simulink model "SIXDOF28"  (R2025b)
settings: Solver=VariableStepAuto  StartTime=0.0  StopTime=sortieStopTime_s  MaxStep=2.0  RelTol=1e-3
undefined symbols (not defined in the file): aircraft_mass, alpha0, alpha_bp, b, CL_table, ClCsurfaces, Cldampingrates, Cldeltae, CmCsurfaces, Cmdampingrates, CnCsurfaces, Cndampingrates, COP, CruiseSpeed, deg, density, DiscIntNeverNeededParam, dwGrad, ElTrim, g, h0, InitialHeadingRadBySortie, InitialPosBySortie, InitPitch, InitUb, Initwb, l, lt, maxPropRad, payloadvolume, PitchTrim, rad, rho, s, S, selectedSortie, St, ThrottleTrim
libraries: slpidlib x12, aerolibasang x3, aerolibconvert2 x2, aerolibadyn x1
(part 3 of 3)

== matlab function SIXDOF28/Subsystem2/Spraying/MATLAB Function2 ==
  settings: updateMethod=DISCRETE
  data: currentPosNED input; sprayActive output; sprayWaypointsNED input; activeSprayLaneIdx output; startGateHit output; endGateHit output; crossTrackToLane_m output; alongTrack_m output; heightError_m output; gateState output; inStartGate output; inEndGate output
function [sprayActive, activeSprayLaneIdx, startGateHit, endGateHit, ...
    crossTrackToLane_m, alongTrack_m, heightError_m, gateState, ...
    inStartGate, inEndGate] = sprayGateLogicNED(currentPosNED, sprayWaypointsNED)
%#codegen
% sprayGateLogicNED
% Simulink-friendly spray on/off logic using rectangular start/end gates
% built from spray-lane start/end waypoint pairs in NED coordinates.
%
% Inputs:
%   currentPosNED      [1x3] or [3x1] vehicle position [North East Down] [m]
%   sprayWaypointsNED  [2*N x 3] spray-lane waypoint pairs:
%                      [start1; end1; start2; end2; ...]
%
% Outputs:
%   sprayActive          1 while spraying on the active lane, else 0
%   activeSprayLaneIdx   current spray lane index being armed or sprayed
%   startGateHit         1 on the sample when the start gate is crossed
%   endGateHit           1 on the sample when the end gate is crossed
%   crossTrackToLane_m   signed horizontal cross-track error to active lane [m]
%   alongTrack_m         along-track position on active lane from lane start [m]
%   heightError_m        vertical error to closest point on active lane [m]
%   gateState            0 waiting for start gate, 1 spraying, 2 complete
%   inStartGate          1 when current position is inside the start gate box
%   inEndGate            1 when current position is inside the end gate box
%
% Gate geometry assumptions:
% - Start and end gates are rectangles perpendicular to the lane direction.
% - Gate width is 10 m total (5 m either side of the lane centreline).
% - Gate thickness is 2 m along the lane direction.
% - Gate height is 2 m total around the planned waypoint altitude.
% - Spray turns on when the aircraft crosses the start gate in the correct
%   direction and within the gate bounds.
% - Spray turns off when the aircraft crosses the end gate in the correct
%   direction and within the gate bounds.

    persistent laneIdxPersistent sprayOnPersistent ...
        previousPosPersistent hasPreviousPosPersistent ...
        previousWaypointCount previousFirstNorth previousFirstEast previousFirstDown ...
        previousLastNorth previousLastEast previousLastDown

    pos = zeros(1,3);
    pos(1) = currentPosNED(1);
    pos(2) = currentPosNED(2);
    pos(3) = currentPosNED(3);

    sprayActive = 0.0;
    activeSprayLaneIdx = 1.0;
    startGateHit = 0.0;
    endGateHit = 0.0;
    crossTrackToLane_m = 0.0;
    alongTrack_m = 0.0;
    heightError_m = 0.0;
    gateState = 0.0;
    inStartGate = 0.0;
    inEndGate = 0.0;

    waypointCount = size(sprayWaypointsNED, 1);
    if waypointCount < 2 || size(sprayWaypointsNED, 2) < 3
        return
    end

    laneCount = floor(waypointCount / 2);
    if laneCount < 1
        return
    end

    if isempty(laneIdxPersistent)
        laneIdxPersistent = 1;
        sprayOnPersistent = false;
        previousPosPersistent = pos;
        hasPreviousPosPersistent = false;
        previousWaypointCount = waypointCount;
        previousFirstNorth = sprayWaypointsNED(1,1);
        previousFirstEast = sprayWaypointsNED(1,2);
        previousFirstDown = sprayWaypointsNED(1,3);
        previousLastNorth = sprayWaypointsNED(waypointCount,1);
        previousLastEast = sprayWaypointsNED(waypointCount,2);
        previousLastDown = sprayWaypointsNED(waypointCount,3);
    end

    if previousWaypointCount ~= waypointCount || ...
            previousFirstNorth ~= sprayWaypointsNED(1,1) || ...
            previousFirstEast ~= sprayWaypointsNED(1,2) || ...
            previousFirstDown ~= sprayWaypointsNED(1,3) || ...
            previousLastNorth ~= sprayWaypointsNED(waypointCount,1) || ...
            previousLastEast ~= sprayWaypointsNED(waypointCount,2) || ...
            previousLastDown ~= sprayWaypointsNED(waypointCount,3)
        laneIdxPersistent = 1;
        sprayOnPersistent = false;
        previousPosPersistent = pos;
        hasPreviousPosPersistent = false;
        previousWaypointCount = waypointCount;
        previousFirstNorth = sprayWaypointsNED(1,1);
        previousFirstEast = sprayWaypointsNED(1,2);
        previousFirstDown = sprayWaypointsNED(1,3);
        previousLastNorth = sprayWaypointsNED(waypointCount,1);
        previousLastEast = sprayWaypointsNED(waypointCount,2);
        previousLastDown = sprayWaypointsNED(waypointCount,3);
    end

    gateHalfWidth_m = 30.0;
    gateHalfThickness_m = 3.0;
    gateHalfHeight_m = 20.0;

    laneIdxForDebug = min(max(laneIdxPersistent, 1), laneCount);
    rowStart = 2 * laneIdxForDebug - 1;
    rowEnd = 2 * laneIdxForDebug;
    laneStartNED = sprayWaypointsNED(rowStart, :);
    laneEndNED = sprayWaypointsNED(rowEnd, :);

    [laneValid, laneUnitNE, laneNormalNE, laneLength_m] = ...
        computeLaneBasis(laneStartNED, laneEndNED);

    if ~laneValid
        if laneIdxPersistent < laneCount
            laneIdxPersistent = laneIdxPersistent + 1;
            previousPosPersistent = pos;
            hasPreviousPosPersistent = true;
            activeSprayLaneIdx = laneIdxPersistent;
            gateState = double(sprayOnPersistent);
        else
            sprayOnPersistent = false;
            laneIdxPersistent = laneCount + 1;
            activeSprayLaneIdx = laneIdxPersistent;
            gateState = 2.0;
        end
        return
    end

    [crossTrackToLane_m, alongTrack_m, heightError_m] = ...
        computeLaneTrackingDebug(pos, laneStartNED, laneEndNED, laneUnitNE, laneNormalNE, laneLength_m);

    startAlongCurrent_m = dot2(pos(1:2) - laneStartNED(1:2), laneUnitNE);
    startCrossCurrent_m = dot2(pos(1:2) - laneStartNED(1:2), laneNormalNE);
    startHeightErrorCurrent_m = pos(3) - laneStartNED(3);
    inStartGate = double(abs(startAlongCurrent_m) <= gateHalfThickness_m && ...
        abs(startCrossCurrent_m) <= gateHalfWidth_m && ...
        abs(startHeightErrorCurrent_m) <= gateHalfHeight_m);

    endAlongCurrent_m = dot2(pos(1:2) - laneEndNED(1:2), laneUnitNE);
    endCrossCurrent_m = dot2(pos(1:2) - laneEndNED(1:2), laneNormalNE);
    endHeightErrorCurrent_m = pos(3) - laneEndNED(3);
    inEndGate = double(abs(endAlongCurrent_m) <= gateHalfThickness_m && ...
        abs(endCrossCurrent_m) <= gateHalfWidth_m && ...
        abs(endHeightErrorCurrent_m) <= gateHalfHeight_m);

    if hasPreviousPosPersistent
        prevPos = previousPosPersistent;
    else
        prevPos = pos;
    end

    if laneIdxPersistent <= laneCount && hasPreviousPosPersistent
        if ~sprayOnPersistent
            startGateHit = double(checkGateCrossing(prevPos, pos, laneStartNED, laneUnitNE, laneNormalNE, ...
                gateHalfWidth_m, gateHalfHeight_m));
            if startGateHit > 0.5
                sprayOnPersistent = true;
            end
        else
            endGateHit = double(checkGateCrossing(prevPos, pos, laneEndNED, laneUnitNE, laneNormalNE, ...
                gateHalfWidth_m, gateHalfHeight_m));
            if endGateHit > 0.5
                sprayOnPersistent = false;
                if laneIdxPersistent < laneCount
                    laneIdxPersistent = laneIdxPersistent + 1;
                else
                    laneIdxPersistent = laneCount + 1;
                end
            end
        end
    end

    sprayActive = double(sprayOnPersistent);
    activeSprayLaneIdx = laneIdxPersistent;

    if laneIdxPersistent > laneCount
        sprayActive = 0.0;
        gateState = 2.0;
    elseif sprayOnPersistent
        gateState = 1.0;
    else
        gateState = 0.0;
    end

    previousPosPersistent = pos;
    hasPreviousPosPersistent = true;
end

function [laneValid, laneUnitNE, laneNormalNE, laneLength_m] = computeLaneBasis(laneStartNED, laneEndNED)
    laneVecNE = laneEndNED(1:2) - laneStartNED(1:2);
    laneLength_m = hypot(laneVecNE(1), laneVecNE(2));
    laneUnitNE = [1.0 0.0];
    laneNormalNE = [0.0 1.0];
    laneValid = laneLength_m > 1e-9;

    if laneValid
        laneUnitNE = laneVecNE / laneLength_m;
        laneNormalNE = [laneUnitNE(2), -laneUnitNE(1)];
    end
end

function [crossTrackToLane_m, alongTrack_m, heightError_m] = ...
    computeLaneTrackingDebug(posNED, laneStartNED, laneEndNED, laneUnitNE, laneNormalNE, laneLength_m)
    deltaNE = posNED(1:2) - laneStartNED(1:2);
    alongTrack_m = dot2(deltaNE, laneUnitNE);
    crossTrackToLane_m = dot2(deltaNE, laneNormalNE);

    alongTrackClamped_m = min(max(alongTrack_m, 0.0), laneLength_m);
    if laneLength_m <= 1e-9
        closestPointD = laneStartNED(3);
    else
        alpha = alongTrackClamped_m / laneLength_m;
        closestPointD = laneStartNED(3) + alpha * (laneEndNED(3) - laneStartNED(3));
    end

    heightError_m = posNED(3) - closestPointD;
end

function crossed = checkGateCrossing(prevPosNED, currPosNED, gateCenterNED, laneUnitNE, laneNormalNE, ...
    gateHalfWidth_m, gateHalfHeight_m)
    crossed = false;

    prevAlong_m = dot2(prevPosNED(1:2) - gateCenterNED(1:2), laneUnitNE);
    currAlong_m = dot2(currPosNED(1:2) - gateCenterNED(1:2), laneUnitNE);

    if ~isfinite(prevAlong_m) || ~isfinite(currAlong_m)
        return
    end

    deltaAlong_m = currAlong_m - prevAlong_m;
    if deltaAlong_m <= 1e-9
        return
    end

    if prevAlong_m > 0.0 || currAlong_m < 0.0
        return
    end

    denom = prevAlong_m - currAlong_m;
    if abs(denom) <= 1e-12
        alpha = 0.0;
    else
        alpha = prevAlong_m / denom;
    end

    alpha = min(max(alpha, 0.0), 1.0);
    intersectPosNED = prevPosNED + alpha * (currPosNED - prevPosNED);

    crossTrackAtCrossing_m = dot2(intersectPosNED(1:2) - gateCenterNED(1:2), laneNormalNE);
    heightErrorAtCrossing_m = intersectPosNED(3) - gateCenterNED(3);

    crossed = abs(crossTrackAtCrossing_m) <= gateHalfWidth_m && ...
        abs(heightErrorAtCrossing_m) <= gateHalfHeight_m;
end

function out = dot2(a, b)
    out = a(1) * b(1) + a(2) * b(2);
end

== matlab function SIXDOF28/Subsystem2/Spraying/MATLAB Function3 ==
  data: spraySignal input; massDot_kgps output; massFlowRelVel_b_mps output
function [massDot_kgps, massFlowRelVel_b_mps] = sprayMassDerivative(spraySignal)
%#codegen
% sprayMassDerivative
% Returns the vehicle mass derivative [kg/s] and mass-flow relative
% velocity [m/s] in body axes from a binary spray command.
% When spraySignal is 1, mass decreases at 0.2025 kg/s and the relative
% velocity is 5 m/s downward in body axes.

    if spraySignal > 0.5
        massDot_kgps = -0.2322;
        massFlowRelVel_b_mps = [0.0; 0.0; 5.0];
    else
        massDot_kgps = 0.0;
        massFlowRelVel_b_mps = [0.0; 0.0; 0.0];
    end
end
